simulink model "FirstPart_TimeFreqSimulink"  (R2026a)
settings: Solver=VariableStepAuto  StopTime=20
libraries: dspxfrm3 x1, dspvision x1
settings Model: Creator=YazanK  LastModifiedBy=pc

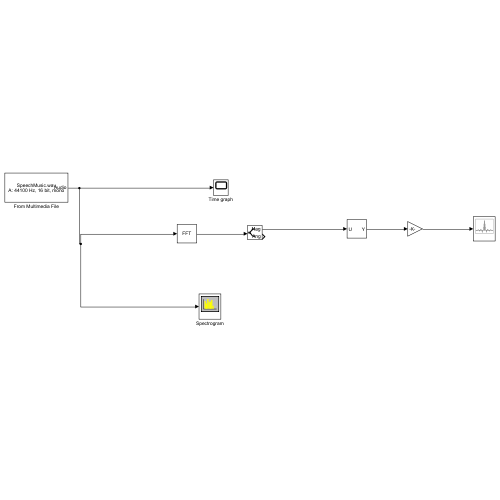
[thumbnail: Simulink's stored preview of the top-level diagram]
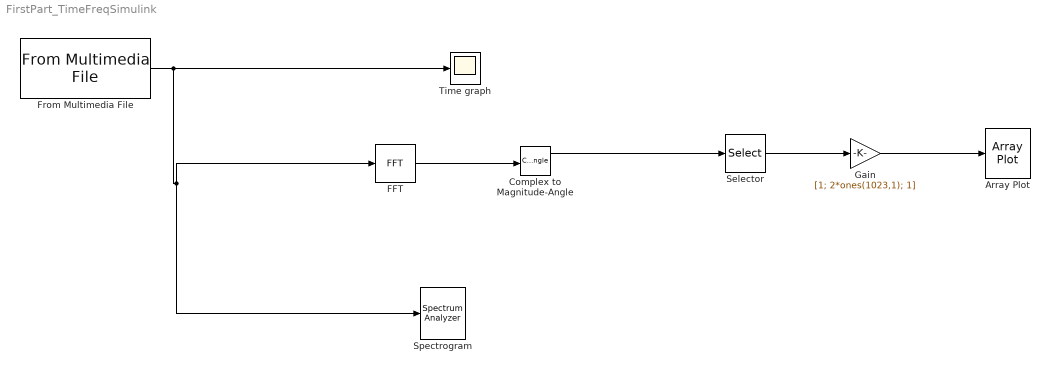
== system FirstPart_TimeFreqSimulink ==
  Array Plot : ArrayPlot  WindowPosition=[261.000000,127.000000,808.000000,611.000000,]  ScopeFrameLocation=window  SampleIncrement=21.533203125  YLimits=[-0.0026 0.023]
  Complex to Magnitude-Angle : ComplexToMagnitudeAngle
  FFT : dspxfrm3/FFT  FFTImplementation=Auto  CompMethod=Table lookup  TableOpt=NEW  TableOptActive=Speed  BitRevOrder=off  Normalize=on  InheritFFTLength=on  FFTLength=64  WrapInput=on  roundingMode=Ceiling  overflowMode=off  firstCoeffDataTypeStr=Inherit: Same word length as input  firstCoeffLastDataTypeStr=Inherit: Same word length as input  outputMin=[]  outputMax=[]
  From Multimedia File : dspvision/From Multimedia File  inputFilename=Audios/SpeechMusic.wav  readRange=[1 Inf]  loop=on  numPlays=inf  outputStreams=Audio only  videoDataType=single  audioDataType=double  inheritSampleTime=on  userDefinedSampleTime=1/30  noAudioOutput=off  isIntensityVideo=off  fourcc=RGB  colorVideoFormat=One multidimensional signal  outputEOF=off  dataOrg=Column-major  audioFrameSize=2048  computeAudioFrameSize=off  outSamplingMode=Sample based
      settings: LibrarySourceBlock=dspsrcs4/From Multimedia File
  Gain : Gain  Gain=[1; 2*ones(1023,1); 1]
  Selector : Selector  InputPortWidth=2048  IndexOptions=Index vector (dialog)  Indices=1:1025  OutputSizes=1
  Spectrogram : SpectrumAnalyzer  WindowPosition=[65.000000,-13.000000,958.000000,844.000000,]  ScopeFrameLocation=window  SpectrumType=Power density  ViewType=Spectrogram  Method=Welch  PlotAsTwoSidedSpectrum=off  FrequencyResolutionMethod=Window length  WindowInvariantSamplesPerUpdate=on  WindowLength=1323  FFTLengthSource=Property  FFTLength=2048  Span=22050  CenterFrequency=11025  StartFrequency=0  StopFrequency=22050  Window=Hamming  OverlapPercent=66.7  SpectrumUnits=dBW/Hz  TimeOrientation=Horizontal  TimeSpanSource=Property  TimeSpan=20  MaximizeAxes=Off  YLimits=[-120.8854793133496 7.496120686650402]  ColorLimits=[-135.33055 -29.49384]  AxesLayout=Horizontal  SelectedToolstripTab=spectrumAnalyzerToolstrip.estimationTab  DataDisplayPrecision=5
  Time graph : Scope
      settings: TimeUnits=Metric (based on Time Span)  ActiveDisplayYMinimum=0.03961341442844174  ActiveDisplayYMaximum=0.0895636045639299  YLabel=Amplitude
  wires:
  From Multimedia File/1 -> Spectrogram/1, FFT/1, Time graph/1
  FFT/1 -> Complex to Magnitude-Angle/1
  Complex to Magnitude-Angle/1 -> Selector/1
  Selector/1 -> Gain/1
  Gain/1 -> Array Plot/1
